simulink model "sm_trackV_lib_chain_lower_frame_s46i1u2l7_ptcld_planar"  (R2026b)
settings: Solver=VariableStepAuto
undefined symbols (not defined in the file): Excv, Right, track_joint_targets, X, Y, Z
libraries: sm_lib x4, sm_trackV_lib_chain_contact x3, sm_trackV_lib_chain_track_s46 x1, sm_trackV_lib_chain_underc_i1u2l7 x1
settings Model: Creator=smiller  LastModifiedBy=smiller

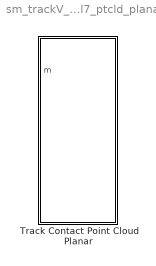
== system sm_trackV_lib_chain_lower_frame_s46i1u2l7_ptcld_planar ==
  Track Contact Point Cloud Planar : Subsystem  mask(Lower Frame with Point Cloud Contact (Planar)){popup_leftOrRight=Right, sprk_xc=Excv.Sprocket.sprocket_xc, sprk_len=Excv.Sprocket.sprk_width, sprk_rho=Excv.Sprocket.density, sprk_clr=Excv.Sprocket.clr, sprk_opc=Excv.Sprocket.opc, sprk_contact_geo_ptcld=Excv.Sprocket.teeth_contact.ptcld.pts(:,1:2), sprk_contact_geo_rad=Excv.Sprocket.teeth_contact.ptcld.rad, sprk_contact_geo_clr=Excv.Sprocket.teeth_contact.ptcld.clr, sprk_contact_geo_opc=Excv.Sprocket.teeth_contact.ptcld.opc, idler_rad=Excv.Idler.rad, idler_len=Excv.Idler.len, idler_rho=Excv.Idler.rho, idler_clr=Excv.Idler.clr, idler_opc=Excv.Idler.opc, idler_contgeo_clr=Excv.Idler.chain_contact.clr, idler_contgeo_opc=Excv.Idler.chain_contact.opc, roller_upper_rad=Excv.Roller.Upper.rad, roller_upper_len=Excv.Roller.Upper.len, roller_upper_rho=Excv.Roller.Upper.rho, roller_upper_clr=Excv.Roller.Upper.clr, roller_upper_opc=Excv.Roller.Upper.opc, roller_upper_contgeo_clr=[1.0 0.0 0.0], roller_upper_contgeo_opc=1, roller_lower_rad=Excv.Roller.Lower.rad, roller_lower_len=Excv.Roller.Lower.len, roller_lower_rho=Excv.Roller.Lower.rho, roller_lower_clr=Excv.Roller.Lower.clr, roller_lower_opc=Excv.Roller.Lower.opc, roller_lower_contgeo_clr=[1.0 0.0 0.0], roller_lower_contgeo_opc=1, tensioner_cyl_len=Excv.Idler.Tensioner.cyl.len, tensioner_cyl_rad=Excv.Idler.Tensioner.cyl.rad, tensioner_cyl_rho=Excv.Idler.Tensioner.cyl.rho, tensioner_cyl_clr=Excv.Idler.Tensioner.cyl.clr, tensioner_cyl_opc=Excv.Idler.Tensioner.cyl.opc, tensioner_pist_len=Excv.Idler.Tensioner.piston.len, tensioner_pist_rad=Excv.Idler.Tensioner.piston.rad, tensioner_pist_rho=Excv.Idler.Tensioner.piston.rho, tensioner_pist_clr=Excv.Idler.Tensioner.piston.clr, tensioner_pist_opc=Excv.Idler.Tensioner.piston.opc, tensioner_br_length=Excv.Idler.Tensioner.bracket.len, tensioner_br_width=Excv.Idler.Tensioner.bracket.wid, tensioner_br_height=Excv.Idler.Tensioner.bracket.height, tensioner_br_thk=Excv.Idler.Tensioner.bracket.thk, tensioner_br_rho=Excv.Idler.Tensioner.bracket.rho, tensioner_br_clr=Excv.Idler.Tensioner.bracket.clr, tensioner_br_opc=Excv.Idler.Tensioner.bracket.opc, tensioner_eqpos=Excv.Idler.Tensioner.xeq, tensioner_x0=Excv.Idler.Tensioner.x0, tensioner_k=Excv.Idler.Tensioner.K, tensioner_b=Excv.Idler.Tensioner.B, roller_upper_x=Excv.Frame.Sprk2UpperX, roller_lower_x=Excv.Frame.Sprk2LowerX, idler_x=Excv.Frame.IdlerAssyX, axle_x=Excv.Frame.AxleX, roller_upper_y=Excv.Frame.Sprk2UpperY, roller_lower_y=Excv.Frame.Sprk2LowerY, idler_y=Excv.Frame.Sprk2IdlerY, axle_y=Excv.Frame.AxleY, sprk_pitch_rad=Excv.Sprocket.sprocket_rPitch, frame_cg_offset=Excv.Frame.CGOffset, frame_mass=Excv.Frame.Mass, frame_moi=Excv.Frame.MOI, frame_poi=Excv.Frame.POI, frame_susp_offset=Excv.Frame.SuspOffset, chain_wid=Excv.Chain.chain_wid, chain_seg_m=Excv.Chain.link_m, chain_seg_cg=Excv.Chain.link_cg, chain_seg_moi=Excv.Chain.link_moi, chain_seg_poi=Excv.Chain.link_poi, plate_xc=Excv.Chain.plate_xc, plate_h=Excv.Chain.plate_h, pin_sep=Excv.Chain.pin_sep, plate_thk=Excv.Chain.plate_thk, plate_ang=Excv.Chain.plate_ang, plate_clr=Excv.Chain.plate_clr, plate_opc=Excv.Chain.plate_opc, pin_len=Excv.Chain.pin_len, pin_rad=Excv.Chain.pin_rad, pin_clr=Excv.Chain.pin_clr, pin_opc=Excv.Chain.pin_opc, shoe_xc=Excv.Shoe.xc, shoe_w=Excv.Shoe.w, shoe_m=Excv.Shoe.mass, shoe_cg=Excv.Shoe.cg, shoe_moi=Excv.Shoe.moi, shoe_poi=Excv.Shoe.poi, shoe_clr=Excv.Shoe.clr, shoe_opc=Excv.Shoe.opc, jointTargets=track_joint_targets, chainDamping=Excv.Chain.damping, ptcld_shoe=Excv.Shoe.ground_contact.ptcld.pts, ptcld_shoe_rad=Excv.Shoe.ground_contact.ptcld.rad, ptcld_shoe_clr=Excv.Shoe.ground_contact.ptcld.clr, ptcld_shoe_opc=Excv.Shoe.ground_contact.ptcld.opc, chain_to_roller_clr=Excv.Chain.roller_contact.clr, chain_to_roller_opc=Excv.Chain.roller_contact.opc, chain_to_teeth_clr=Excv.Chain.teeth_contact.clr, chain_to_teeth_opc=Excv.Chain.teeth_contact.opc, B_Sprocket=Excv.Contact.Sprocket.B, K_Sprocket=Excv.Contact.Sprocket.K, TW_Sprocket=Excv.Contact.Sprocket.TW, K_Roller=Excv.Contact.Roller.K, B_Roller=Excv.Contact.Roller.B, TW_Roller=Excv.Contact.Roller.TW, K_Idler=Excv.Contact.Idler.K, B_Idler=Excv.Contact.Idler.B, TW_Idler=Excv.Contact.Idler.TW, popup_sense_roller=Constraint Force}
      mask prompts: popup_leftOrRight "Left or Right"; sprk_xc "Extrusion Data [x y] (m)"; sprk_len "Length (m)"; sprk_rho "Density (kg/m^3)"; sprk_clr "Color [R G B] (0-1)"; sprk_opc "Opacity (0-1)"; sprk_contact_geo_ptcld "Point Cloud Data [x y z] (m)"; sprk_contact_geo_rad "Radius (m)"; sprk_contact_geo_clr "Color [R G B] (0-1)"; sprk_contact_geo_opc "Opacity (0-1)"; idler_rad "Idler Radius (m)"; idler_len "Length (m)"; idler_rho "Density (kg/m^3)"; idler_clr "Color [R G B] (0-1)"; idler_opc "Opacity (0-1)"; idler_contgeo_clr "Color [R G B] (0-1)"; idler_contgeo_opc "Opacity (0-1)"; roller_upper_rad "Radius (m)"; roller_upper_len "Length (m)"; roller_upper_rho "Density (kg/m^3)"; roller_upper_clr "Color [R G B] (0-1)"; roller_upper_opc "Opacity (0-1)"; roller_upper_contgeo_clr "Color [R G B] (0-1)"; roller_upper_contgeo_opc "Opacity (0-1)"; roller_lower_rad "Lower Roller Radius (m)"; roller_lower_len "Length (m)"; roller_lower_rho "Density (kg/m^3)"; roller_lower_clr "Color [R G B] (0-1)"; roller_lower_opc "Opacity (0-1)"; roller_lower_contgeo_clr "Color [R G B] (0-1)"; roller_lower_contgeo_opc "Opacity (0-1)"; tensioner_cyl_len "Length (m)"; tensioner_cyl_rad "Radius (m)"; tensioner_cyl_rho "Density (kg/m^3)"; tensioner_cyl_clr "Color [R G B] (0-1)"; tensioner_cyl_opc "Opacity (0-1)"; tensioner_pist_len "Length (m)"; tensioner_pist_rad "Radius (m)"; tensioner_pist_rho "Density (kg/m^3)"; tensioner_pist_clr "Color [R G B] (0-1)"; tensioner_pist_opc "Opacity (0.1)"; tensioner_br_length "Length (m)"; tensioner_br_width "Width (m)"; tensioner_br_height "Height (m)"; tensioner_br_thk "Thickness (m)"; tensioner_br_rho "Density (kg/m^3)"; tensioner_br_clr "Color [R G B] (0-1)"; tensioner_br_opc "Opacity (0-1)"; tensioner_eqpos "Equilibrium Position (m)"; tensioner_x0 "Assembly Position (m)"; tensioner_k "Stiffness Coefficient (N/m)"; tensioner_b "Damping Coefficient (N/(m/s))"; roller_upper_x "Upper Rollers (vector) (m)"; roller_lower_x "Lower Rollers (vector) (m)"; idler_x "Idler Wheel (m)"; axle_x "Axle (m)"; roller_upper_y "Sprocket to Upper Rollers (m)"; roller_lower_y "Sprocket to Lower Rollers (m)"; idler_y "Sprocket to Idler (m)"; axle_y "Sprocket to Axle (m)"; sprk_pitch_rad "Sprocket Pitch Radius (m)"; frame_cg_offset "CG Offset from Sprocket [x y z] (m)"; frame_mass "Mass (kg)"; frame_moi "Moments of Inertia [Ixx Iyy Izz] (kg*m^2)"; frame_poi "Products of Inertia [Ixx Iyy Izz] (kg*m^2)"; frame_susp_offset "Suspension Offset from Sprocket [x y z] (m)"; chain_wid "Width (m)"; chain_seg_m "Mass (kg)"; chain_seg_cg "CG [x y z] (kg)"; chain_seg_moi "Moments of Inertia [Ixx Iyy Izz] (kg*m^2)"; chain_seg_poi "Products of Inertia [Iyz Ixz Ixy] (kg*m^2)"; plate_xc "Extrusion [x y] (m)"; plate_h "Height (m)"; pin_sep "Pin Separation (m)"; plate_thk "Thickness (m)"; plate_ang "Angle (deg)"; plate_clr "Color [R G B] (0-1)"; plate_opc "Opacity (0-1)"; pin_len "Pin Length (m)"; pin_rad "Pin Radius (m)"; pin_clr "Pin Color [R G B] (0-1)"; pin_opc "Opacity (0-1)"; shoe_xc "Extrusion Profile [x y] (m)"; shoe_w "Width (m)"; shoe_m "Mass (kg)"; shoe_cg "CG [x y z ] (m)"; shoe_moi "Moments of Inertia [Ixx Iyy Izz] (kg*m^2)"; shoe_poi "Products of Inertia [Iyz Izx Ixy] (kg*m^2)"; shoe_clr "Color [R G B] (0-1)"; shoe_opc "Opacity (0-1)"; jointTargets "Joint Targets (structure)"; chainDamping "Joint Damping N*m/(deg/s)"; ptcld_shoe "Points [x y z] (m)"; ptcld_shoe_rad "Radius (m)"; ptcld_shoe_clr "Color [R G B] (0-1)"; ptcld_shoe_opc "Opacity (0-1)"; chain_to_roller_clr "Color [R G B] (0-1)"; chain_to_roller_opc "Opacity (0-1)"; chain_to_teeth_clr "Color [R G B] (0-1)"; chain_to_teeth_opc "Opacity (0-1)"; B_Sprocket "Normal Damping (N/(m/s))"; K_Sprocket "Normal Stiffness (N/m)"; TW_Sprocket "Normal Transition Width (m)"; K_Roller "Normal Stiffness (N/m)"; B_Roller "Normal Damping (N/(m/s))"; TW_Roller "Normal Transition Width (m)"; K_Idler "Normal Stiffness (N/m)"; B_Idler "Normal Damping (N/(m/s))"; TW_Idler "Normal Transition Width (m)"; popup_sense_roller "Roller"
      mask help: Models a segmented track with undercarriage. Contact geometry (point cloud) in track segment shoes enable contact with the ground. Includes sprocket, rollers, and idler with tensioner. Contact forces within the track are planar to speed up simulation. The sprocket has a 1D rotational mechanical interface to the drivetrain.
      mask init:
      | bh = gcb;
      | set_param([bh '/Undercarriage'],'popup_sense_roller',get_param(bh,'popup_sense_roller'));
      mask TypeOptions popup_leftOrRight: Undercarriage/popup_leftOrRight
      mask TypeOptions sprk_xc: Undercarriage/sprk_xc
      mask TypeOptions sprk_len: Undercarriage/sprk_len
      mask TypeOptions sprk_rho: Undercarriage/sprk_rho
      mask TypeOptions sprk_clr: Undercarriage/sprk_clr
      mask TypeOptions sprk_opc: Undercarriage/sprk_opc
      mask TypeOptions sprk_contact_geo_ptcld: Undercarriage/sprk_contact_geo_ptcld
      mask TypeOptions sprk_contact_geo_rad: Undercarriage/sprk_contact_geo_rad
      mask TypeOptions sprk_contact_geo_clr: Undercarriage/sprk_contact_geo_clr
      mask TypeOptions sprk_contact_geo_opc: Undercarriage/sprk_contact_geo_opc
      mask TypeOptions idler_rad: Undercarriage/idler_rad
      mask TypeOptions idler_len: Undercarriage/idler_len
      mask TypeOptions idler_rho: Undercarriage/idler_rho
      mask TypeOptions idler_clr: Undercarriage/idler_clr
      mask TypeOptions idler_opc: Undercarriage/idler_opc
      mask TypeOptions idler_contgeo_clr: Undercarriage/idler_contgeo_clr
      mask TypeOptions idler_contgeo_opc: Undercarriage/idler_contgeo_opc
      mask TypeOptions roller_upper_rad: Undercarriage/roller_upper_rad
      mask TypeOptions roller_upper_len: Undercarriage/roller_upper_len
      mask TypeOptions roller_upper_rho: Undercarriage/roller_upper_rho
      mask TypeOptions roller_upper_clr: Undercarriage/roller_upper_clr
      mask TypeOptions roller_upper_opc: Undercarriage/roller_upper_opc
      mask TypeOptions roller_upper_contgeo_clr: Undercarriage/roller_upper_contgeo_clr
      mask TypeOptions roller_upper_contgeo_opc: Undercarriage/roller_upper_contgeo_opc
      mask TypeOptions roller_lower_rad: Undercarriage/roller_lower_rad
      mask TypeOptions roller_lower_len: Undercarriage/roller_lower_len
      mask TypeOptions roller_lower_rho: Undercarriage/roller_lower_rho
      mask TypeOptions roller_lower_clr: Undercarriage/roller_lower_clr
      mask TypeOptions roller_lower_opc: Undercarriage/roller_lower_opc
      mask TypeOptions roller_lower_contgeo_clr: Undercarriage/roller_lower_contgeo_clr
      mask TypeOptions roller_lower_contgeo_opc: Undercarriage/roller_lower_contgeo_opc
      mask TypeOptions tensioner_cyl_len: Undercarriage/tensioner_cyl_len
      mask TypeOptions tensioner_cyl_rad: Undercarriage/tensioner_cyl_rad
      mask TypeOptions tensioner_cyl_rho: Undercarriage/tensioner_cyl_rho
      mask TypeOptions tensioner_cyl_clr: Undercarriage/tensioner_cyl_clr
      mask TypeOptions tensioner_cyl_opc: Undercarriage/tensioner_cyl_opc
      mask TypeOptions tensioner_pist_len: Undercarriage/tensioner_pist_len
      mask TypeOptions tensioner_pist_rad: Undercarriage/tensioner_pist_rad
      mask TypeOptions tensioner_pist_rho: Undercarriage/tensioner_pist_rho
      mask TypeOptions tensioner_pist_clr: Undercarriage/tensioner_pist_clr
      mask TypeOptions tensioner_pist_opc: Undercarriage/tensioner_pist_opc
      mask TypeOptions tensioner_br_length: Undercarriage/tensioner_br_length
      mask TypeOptions tensioner_br_width: Undercarriage/tensioner_br_width
      mask TypeOptions tensioner_br_height: Undercarriage/tensioner_br_height
      mask TypeOptions tensioner_br_thk: Undercarriage/tensioner_br_thk
      mask TypeOptions tensioner_br_rho: Undercarriage/tensioner_br_rho
      mask TypeOptions tensioner_br_clr: Undercarriage/tensioner_br_clr
      mask TypeOptions tensioner_br_opc: Undercarriage/tensioner_br_opc
      mask TypeOptions tensioner_eqpos: Undercarriage/tensioner_eqpos
      mask TypeOptions tensioner_x0: Undercarriage/tensioner_x0
      mask TypeOptions tensioner_k: Undercarriage/tensioner_k
      mask TypeOptions tensioner_b: Undercarriage/tensioner_b
      mask TypeOptions roller_upper_x: Undercarriage/roller_upper_x
      mask TypeOptions roller_lower_x: Undercarriage/roller_lower_x
      mask TypeOptions idler_x: Undercarriage/idler_x
      mask TypeOptions axle_x: Undercarriage/axle_x
      mask TypeOptions roller_upper_y: Undercarriage/roller_upper_y
      mask TypeOptions roller_lower_y: Undercarriage/roller_lower_y
      mask TypeOptions idler_y: Undercarriage/idler_y
      mask TypeOptions axle_y: Undercarriage/axle_y
      mask TypeOptions sprk_pitch_rad:
      | Transform
      | Track/TranslationStandardOffset
      mask TypeOptions frame_cg_offset: Undercarriage/frame_cg_offset
      mask TypeOptions frame_mass: Undercarriage/frame_mass
      mask TypeOptions frame_moi: Undercarriage/frame_moi
      mask TypeOptions frame_poi: Undercarriage/frame_poi
      mask TypeOptions frame_susp_offset: Undercarriage/frame_susp_offset
      mask TypeOptions chain_wid: Track/chain_wid
      mask TypeOptions chain_seg_m: Track/chain_seg_m
      mask TypeOptions chain_seg_cg: Track/chain_seg_cg
      mask TypeOptions chain_seg_moi: Track/chain_seg_moi
      mask TypeOptions chain_seg_poi: Track/chain_seg_poi
      mask TypeOptions plate_xc: Track/plate_xc
      mask TypeOptions plate_h: Track/plate_h
      mask TypeOptions pin_sep: Track/pin_sep
      mask TypeOptions plate_thk: Track/plate_thk
      mask TypeOptions plate_ang: Track/plate_ang
      mask TypeOptions plate_clr: Track/plate_clr
      mask TypeOptions plate_opc: Track/plate_opc
      mask TypeOptions pin_len: Track/pin_len
      mask TypeOptions pin_rad: Track/pin_rad
      mask TypeOptions pin_clr: Track/pin_clr
      mask TypeOptions pin_opc: Track/pin_opc
      mask TypeOptions shoe_xc: Track/shoe_xc
      mask TypeOptions shoe_w: Track/shoe_w
      mask TypeOptions shoe_m: Track/shoe_m
      mask TypeOptions shoe_cg: Track/shoe_cg
      mask TypeOptions shoe_moi: Track/shoe_moi
      mask TypeOptions shoe_poi: Track/shoe_poi
      mask TypeOptions shoe_clr: Track/shoe_clr
      mask TypeOptions shoe_opc: Track/shoe_opc
      mask TypeOptions jointTargets: Track/jointTargets
      mask TypeOptions chainDamping: Track/chainDamping
      mask TypeOptions ptcld_shoe: Track/ptcld_shoe
      mask TypeOptions ptcld_shoe_rad: Track/ptcld_shoe_rad
      mask TypeOptions ptcld_shoe_clr: Track/ptcld_shoe_clr
      mask TypeOptions ptcld_shoe_opc: Track/ptcld_shoe_opc
      mask TypeOptions chain_to_roller_clr: Track/chain_to_roller_clr
      mask TypeOptions chain_to_roller_opc: Track/chain_to_roller_opc
      mask TypeOptions chain_to_teeth_clr: Track/chain_to_teeth_clr
      mask TypeOptions chain_to_teeth_opc: Track/chain_to_teeth_opc
      mask TypeOptions B_Sprocket:
      | CF
      | Chain
      | Sprocket/B_Sprocket
      mask TypeOptions K_Sprocket:
      | CF
      | Chain
      | Sprocket/K_Sprocket
      mask TypeOptions TW_Sprocket:
      | CF
      | Chain
      | Sprocket/TW_Sprocket
      mask TypeOptions K_Roller:
      | CF
      | Chain
      | Rollers/K_Roller
      mask TypeOptions B_Roller:
      | CF
      | Chain
      | Rollers/B_Roller
      mask TypeOptions TW_Roller:
      | CF
      | Chain
      | Rollers/TW_Roller
      mask TypeOptions K_Idler:
      | CF
      | Chain
      | Idler/K_Idler
      mask TypeOptions B_Idler:
      | CF
      | Chain
      | Idler/B_Idler
      mask TypeOptions TW_Idler:
      | CF
      | Chain
      | Idler/TW_Idler
      mask TypeOptions popup_sense_roller: Constraint Force | Actuator Torque
      mask DialogControl cont_sprocket Prompt: Sprocket
      mask DialogControl cont_sprocket_solid Prompt: Solid
      mask DialogControl cont_sprocket_contact_geo Prompt: Contact Geometry
      mask DialogControl cont_idler Prompt: Idler
      mask DialogControl cont_idler_solid Prompt: Solid
      mask DialogControl cont_idler_contact_geo Prompt: Contact Geometry
      mask DialogControl cont_rollers Prompt: Rollers
      mask DialogControl cont_roller_upper Prompt: Upper
      mask DialogControl cont_roller_upper_contact_geo Prompt: Contact Geometry
      mask DialogControl cont_rollers_lower Prompt: Lower
      mask DialogControl cont_rollers_lower_contact_geo Prompt: Contact Geometry
      mask DialogControl cont_tensioner Prompt: Tensioner
      mask DialogControl cont_tensioner_cyl Prompt: Cylinder
      mask DialogControl cont_tensioner_pist Prompt: Piston
      mask DialogControl cont_tensioner_brkt Prompt: Bracket
      mask DialogControl cont_tensioner_assembly Prompt: Assembly
      mask DialogControl cont_frame Prompt: Frame
      mask DialogControl cont_offset_x Prompt: Longitudinal Offsets from Sprocket
      mask DialogControl cont_offset_y Prompt: Vertical Offsets
      mask DialogControl cont_mass Prompt: Mass and Inertia
      mask DialogControl cont_susp Prompt: Suspension Offset
      mask DialogControl cont_chain Prompt: Chain
      mask DialogControl cont_seg Prompt: Segment
      mask DialogControl cont_plates Prompt: Plates
      mask DialogControl cont_pin Prompt: Pin
      mask DialogControl cont_shoe Prompt: Shoe
      mask DialogControl cont_track_assembly Prompt: Assembly
      mask DialogControl cont_contact_geo Prompt: Contact Geometry
      mask DialogControl cont_shoe_ptcld Prompt: Shoe Point Cloud
      mask DialogControl cont_chain_to_roller Prompt: Chain to Roller
      mask DialogControl cont_chain_to_teeth Prompt: Chain to Teeth
      mask DialogControl cont_contact_underc_track Prompt: Contact
      mask DialogControl cont_sensing Prompt: Sensing
      mask Display:
      | image('sm_excv_track_track_topview_IMAGE.png');
      | color('white')
      | disp('Pla')

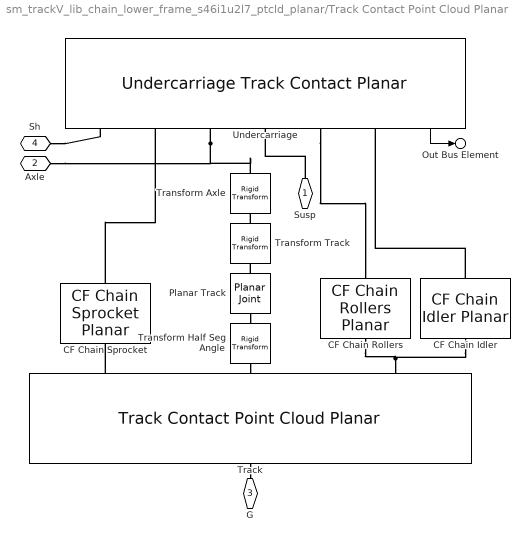
== system sm_trackV_lib_chain_lower_frame_s46i1u2l7_ptcld_planar/Track Contact Point Cloud Planar ==
  CF Chain Idler : sm_trackV_lib_chain_contact/CF Chain Idler Planar  K_Idler=K_Idler  B_Idler=B_Idler  TW_Idler=TW_Idler
  CF Chain Rollers : sm_trackV_lib_chain_contact/CF Chain Rollers Planar  K_Roller=K_Roller  B_Roller=B_Roller  TW_Roller=TW_Roller
  CF Chain Sprocket : sm_trackV_lib_chain_contact/CF Chain Sprocket Planar  K_Sprocket=K_Sprocket  B_Sprocket=B_Sprocket  TW_Sprocket=TW_Sprocket
  Planar Track : sm_lib/Joints/Planar Joint  JointMode=Normal  CompositeWrenchDir=FollowerOnBase  CompositeWrenchFrame=BaseFrame  SenseConstraintForce=off  SenseConstraintTorque=off  SenseTotalForce=off  SenseTotalTorque=off  PxPositionTargetSpecify=on  PxPositionTargetPriority=High  PxPositionTargetValue=0  PxPositionTargetValueUnits=m  PxVelocityTargetSpecify=off  PxVelocityTargetPriority=High  PxVelocityTargetValue=0  PxVelocityTargetValueUnits=m/s  PxEquilibriumPosition=0  PxEquilibriumPositionUnits=m  PxSpringStiffness=0  PxSpringStiffnessUnits=N/m  PxDampingCoefficient=0  PxDampingCoefficientUnits=N/(m/s)  PxLowerLimitSpecify=off  PxLowerLimitBound=-1  PxLowerLimitBoundUnits=m  PxLowerLimitStiffness=1e6  PxLowerLimitStiffnessUnits=N/m  PxLowerLimitDamping=1e3  PxLowerLimitDampingUnits=N/(m/s)  PxLowerLimitTransitionRegionWidth=1e-4  PxLowerLimitTransitionRegionWidthUnits=m  PxUpperLimitSpecify=off  PxUpperLimitBound=1  PxUpperLimitBoundUnits=m  PxUpperLimitStiffness=1e6  PxUpperLimitStiffnessUnits=N/m  PxUpperLimitDamping=1e3  PxUpperLimitDampingUnits=N/(m/s)  PxUpperLimitTransitionRegionWidth=1e-4  PxUpperLimitTransitionRegionWidthUnits=m  PxTorqueActuationMode=NoTorque  PxMotionActuationMode=ComputedMotion  PxSensePosition=off  PxSenseVelocity=off  PxSenseAcceleration=off  PxSenseTorqueForce=off  PxSenseLowerLimitTorqueForce=off  PxSenseUpperLimitTorqueForce=off  PyPositionTargetSpecify=on  PyPositionTargetPriority=High  PyPositionTargetValue=0  PyPositionTargetValueUnits=m  PyVelocityTargetSpecify=off  PyVelocityTargetPriority=High  PyVelocityTargetValue=0  PyVelocityTargetValueUnits=m/s  PyEquilibriumPosition=0  PyEquilibriumPositionUnits=m  PySpringStiffness=0  PySpringStiffnessUnits=N/m  PyDampingCoefficient=0  PyDampingCoefficientUnits=N/(m/s)  PyLowerLimitSpecify=off  PyLowerLimitBound=-1  PyLowerLimitBoundUnits=m  PyLowerLimitStiffness=1e6  PyLowerLimitStiffnessUnits=N/m  PyLowerLimitDamping=1e3  PyLowerLimitDampingUnits=N/(m/s)  PyLowerLimitTransitionRegionWidth=1e-4  PyLowerLimitTransitionRegionWidthUnits=m  PyUpperLimitSpecify=off  PyUpperLimitBound=1  PyUpperLimitBoundUnits=m  PyUpperLimitStiffness=1e6  PyUpperLimitStiffnessUnits=N/m  PyUpperLimitDamping=1e3  PyUpperLimitDampingUnits=N/(m/s)  PyUpperLimitTransitionRegionWidth=1e-4  PyUpperLimitTransitionRegionWidthUnits=m  PyTorqueActuationMode=NoTorque  PyMotionActuationMode=ComputedMotion  PySensePosition=off  PySenseVelocity=off  PySenseAcceleration=off  PySenseTorqueForce=off  PySenseLowerLimitTorqueForce=off  PySenseUpperLimitTorqueForce=off  RzPositionTargetSpecify=off  RzPositionTargetPriority=High  RzPositionTargetValue=0  RzPositionTargetValueUnits=deg  RzVelocityTargetSpecify=off  RzVelocityTargetPriority=High  RzVelocityTargetValue=0  RzVelocityTargetValueUnits=deg/s  RzEquilibriumPosition=0  RzEquilibriumPositionUnits=deg  RzSpringStiffness=0  RzSpringStiffnessUnits=N*m/deg  RzDampingCoefficient=0  RzDampingCoefficientUnits=N*m/(deg/s)  RzLowerLimitSpecify=off  RzLowerLimitBound=-90  RzLowerLimitBoundUnits=deg  RzLowerLimitStiffness=1e4  RzLowerLimitStiffnessUnits=N*m/deg  RzLowerLimitDamping=10  RzLowerLimitDampingUnits=N*m/(deg/s)  RzLowerLimitTransitionRegionWidth=0.1  RzLowerLimitTransitionRegionWidthUnits=deg  RzUpperLimitSpecify=off  RzUpperLimitBound=90  RzUpperLimitBoundUnits=deg  RzUpperLimitStiffness=1e4  RzUpperLimitStiffnessUnits=N*m/deg  RzUpperLimitDamping=10  RzUpperLimitDampingUnits=N*m/(deg/s)  RzUpperLimitTransitionRegionWidth=0.1  RzUpperLimitTransitionRegionWidthUnits=deg  RzTorqueActuationMode=NoTorque  RzMotionActuationMode=ComputedMotion  RzSensePosition=off  RzSenseVelocity=off  RzSenseAcceleration=off  RzSenseTorqueForce=off  RzSenseLowerLimitTorqueForce=off  RzSenseUpperLimitTorqueForce=off
  Track : sm_trackV_lib_chain_track_s46/Track Contact Point Cloud Planar  chain_wid=chain_wid  chain_seg_m=chain_seg_m  chain_seg_cg=chain_seg_cg  chain_seg_moi=chain_seg_moi  chain_seg_poi=chain_seg_poi  plate_h=plate_h  plate_xc=plate_xc  plate_thk=plate_thk  pin_sep=pin_sep  plate_ang=plate_ang  plate_clr=plate_clr  plate_opc=plate_opc  pin_len=pin_len  pin_rad=pin_rad  pin_clr=pin_clr  pin_opc=pin_opc  shoe_xc=shoe_xc  shoe_w=shoe_w  shoe_m=shoe_m  shoe_cg=shoe_cg  shoe_moi=shoe_moi  shoe_poi=shoe_poi  shoe_clr=shoe_clr  shoe_opc=shoe_opc  jointTargets=jointTargets  chainDamping=chainDamping  ptcld_shoe=ptcld_shoe  ptcld_shoe_rad=ptcld_shoe_rad  ptcld_shoe_clr=ptcld_shoe_clr  ptcld_shoe_opc=ptcld_shoe_opc  chain_to_roller_clr=chain_to_roller_clr  chain_to_roller_opc=chain_to_roller_opc  chain_to_teeth_clr=chain_to_teeth_clr  chain_to_teeth_opc=chain_to_teeth_opc
  Transform Axle : sm_lib/Frames and Transforms/Rigid Transform  RotationMethod=None  FollAlignAxisA=+X  BaseAlignAxisA=+Y  FollAlignAxisB=+Y  BaseAlignAxisB=+Z  RotationStandardAxis=+Z  RotationAngle=0.0  RotationAngleUnits=deg  RotationArbitraryAxis=[0 0 1]  RotationSequenceAxes=FollowerAxes  RotationSequence=XYX  RotationSequenceAngles=[0 0 0]  RotationSequenceAnglesUnits=deg  RotationMatrix=[1 0 0; 0 1 0; 0 0 1]  Quaternion=[1 0 0 0]  TranslationMethod=Cartesian  TranslationCartesianOffset=[axle_x -axle_y 0]  TranslationCartesianOffsetUnits=m  TranslationStandardAxis=+X  TranslationStandardOffset=0  TranslationStandardOffsetUnits=m  TranslationROffset=0  TranslationROffsetUnits=m  TranslationThetaOffset=0  TranslationThetaOffsetUnits=deg  TranslationZOffset=0  TranslationZOffsetUnits=m
  Transform Half Seg Angle : sm_lib/Frames and Transforms/Rigid Transform  RotationMethod=StandardAxis  FollAlignAxisA=+X  BaseAlignAxisA=+Y  FollAlignAxisB=+Y  BaseAlignAxisB=+Z  RotationStandardAxis=+Z  RotationAngle=90-acosd(pin_sep/2/sprk_pitch_rad)  RotationAngleUnits=deg  RotationArbitraryAxis=[0 0 1]  RotationSequenceAxes=FollowerAxes  RotationSequence=XYX  RotationSequenceAngles=[0 0 0]  RotationSequenceAnglesUnits=deg  RotationMatrix=[1 0 0; 0 1 0; 0 0 1]  Quaternion=[1 0 0 0]  TranslationMethod=None  TranslationCartesianOffset=[0 0 0]  TranslationCartesianOffsetUnits=m  TranslationStandardAxis=+Z  TranslationStandardOffset=0  TranslationStandardOffsetUnits=m  TranslationROffset=0  TranslationROffsetUnits=m  TranslationThetaOffset=0  TranslationThetaOffsetUnits=deg  TranslationZOffset=0  TranslationZOffsetUnits=m
  Transform Track : sm_lib/Frames and Transforms/Rigid Transform  RotationMethod=StandardAxis  FollAlignAxisA=+X  BaseAlignAxisA=+Y  FollAlignAxisB=+Y  BaseAlignAxisB=+Z  RotationStandardAxis=+Z  RotationAngle=-90  RotationAngleUnits=deg  RotationArbitraryAxis=[0 0 1]  RotationSequenceAxes=FollowerAxes  RotationSequence=XYX  RotationSequenceAngles=[0 0 0]  RotationSequenceAnglesUnits=deg  RotationMatrix=[1 0 0; 0 1 0; 0 0 1]  Quaternion=[1 0 0 0]  TranslationMethod=StandardAxis  TranslationCartesianOffset="[0  0  0]"  TranslationCartesianOffsetUnits=m  TranslationStandardAxis=-X  TranslationStandardOffset=sprk_pitch_rad  TranslationStandardOffsetUnits=m  TranslationROffset=0  TranslationROffsetUnits=m  TranslationThetaOffset=0  TranslationThetaOffsetUnits=deg  TranslationZOffset=0  TranslationZOffsetUnits=m
  Undercarriage : sm_trackV_lib_chain_underc_i1u2l7/Undercarriage Track Contact Planar  popup_leftOrRight=Right  sprk_xc=sprk_xc  sprk_len=sprk_len  sprk_rho=sprk_rho  sprk_clr=sprk_clr  sprk_opc=sprk_opc  sprk_contact_geo_ptcld=sprk_contact_geo_ptcld  sprk_contact_geo_rad=sprk_contact_geo_rad  sprk_contact_geo_clr=sprk_contact_geo_clr  sprk_contact_geo_opc=sprk_contact_geo_opc  idler_rad=idler_rad  idler_len=idler_len  idler_rho=idler_rho  idler_clr=idler_clr  idler_opc=idler_opc  idler_contgeo_clr=idler_contgeo_clr  idler_contgeo_opc=idler_contgeo_opc  roller_upper_rad=roller_upper_rad  roller_upper_len=roller_upper_len  roller_upper_rho=roller_upper_rho  roller_upper_clr=roller_upper_clr  roller_upper_opc=roller_upper_opc  roller_upper_contgeo_clr=roller_upper_contgeo_clr  roller_upper_contgeo_opc=roller_upper_contgeo_opc  roller_lower_rad=roller_lower_rad  roller_lower_len=roller_lower_len  roller_lower_rho=roller_lower_rho  roller_lower_clr=roller_lower_clr  roller_lower_opc=roller_lower_opc  roller_lower_contgeo_clr=roller_lower_contgeo_clr  roller_lower_contgeo_opc=roller_lower_contgeo_opc  tensioner_cyl_len=tensioner_cyl_len  tensioner_cyl_rad=tensioner_cyl_rad  tensioner_cyl_rho=tensioner_cyl_rho  tensioner_cyl_clr=tensioner_cyl_clr  tensioner_cyl_opc=tensioner_cyl_opc  tensioner_pist_len=tensioner_pist_len  tensioner_pist_rad=tensioner_pist_rad  tensioner_pist_rho=tensioner_pist_rho  tensioner_pist_clr=tensioner_pist_clr  tensioner_pist_opc=tensioner_pist_opc  tensioner_br_length=tensioner_br_length  tensioner_br_width=tensioner_br_width  tensioner_br_height=tensioner_br_height  tensioner_br_thk=tensioner_br_thk  tensioner_br_rho=tensioner_br_rho  tensioner_br_clr=tensioner_br_clr  tensioner_br_opc=tensioner_br_opc  tensioner_eqpos=tensioner_eqpos  tensioner_x0=tensioner_x0  tensioner_k=tensioner_k  tensioner_b=tensioner_b  roller_upper_x=roller_upper_x  roller_lower_x=roller_lower_x  idler_x=idler_x  axle_x=axle_x  roller_upper_y=roller_upper_y  roller_lower_y=roller_lower_y  idler_y=idler_y  axle_y=axle_y  frame_cg_offset=frame_cg_offset  frame_mass=frame_mass  frame_moi=frame_moi  frame_poi=frame_poi  frame_susp_offset=frame_susp_offset  popup_sense_roller=Constraint Force
  Susp : PMIOPort  Side=Left
  Axle : PMIOPort  Port=2  Side=Left
  G : PMIOPort  Port=3  Side=Right
  Sh : PMIOPort  Port=4  Side=Right
  Out Bus Element : Outport  PortName=m  Element=Underc
  wires:
  Undercarriage/1 -> Out Bus Element/1
  connections:
  Undercarriage/RConn2 -- CF Chain Rollers/LConn1
  Track/LConn1 -- CF Chain Idler/RConn1 -- CF Chain Rollers/RConn1
  Susp/RConn1 -- Undercarriage/RConn3
  Transform Track/LConn1 -- Transform Axle/LConn1
  Undercarriage/RConn4 -- Transform Axle/RConn1 -- Axle/RConn1
  CF Chain Sprocket/LConn1 -- Undercarriage/RConn5
  Sh/RConn1 -- Undercarriage/RConn6
  Track/LConn3 -- CF Chain Sprocket/RConn1
  CF Chain Idler/LConn1 -- Undercarriage/RConn1
  Track/RConn1 -- G/RConn1
  Planar Track/LConn1 -- Transform Track/RConn1
  Planar Track/RConn1 -- Transform Half Seg Angle/LConn1
  Transform Half Seg Angle/RConn1 -- Track/LConn2
